simulink model "ACC_Controller"  (R2026b)
settings: Solver=FixedStepDiscrete  StopTime=inf  FixedStep=0.05
InitFcn:
  | acc_controller_init;
values from neighbouring files (symbols this model uses):
  C = acc_controller_params()    [acc_controller_init.m]    (also in acc_scenario_input.m; acc_scenarios.m; build_acc_controller.m; replay_mass_estimate.m)
libraries: mpclib x1
settings Model: Creator=kikiw  LastModifiedBy=kikiw
settings OptimizationCC: DefaultParameterBehavior=Inlined  DifferentSizesBufferReuse=on  EfficientTunableParamExpr=on  EnhancedBackFolding=on  OptimizationCustomize=off  OptimizeBlockOrder=speed  PassReuseOutputArgsAs=Individual arguments  RemoveInternalMemoryZeroInit=on  RemoveRootLevelIOMemoryZeroInit=on
settings DebuggingCC: ParameterTunabilityLossMsg=error
settings SFSimCC: MATLABDynamicMemAlloc=off
settings RTWCC: DataTypeReplacement=CDataTypesFixedWidth  Description=Embedded Coder  GenerateReport=on  SystemTargetFile=ert.tlc  TargetLang=C++  TemplateMakefile=ert_default_tmf
settings CodeAppCC: CustomSymbolStrUtil=$R$N$C  ForceParamTrailComments=on  IgnoreCustomStorageClasses=off  InsertBlockDesc=on  OperatorAnnotations=on  SFDataObjDesc=on  SimulinkDataObjDesc=on
settings ERTTargetCC: CodeInterfacePackaging=C++ class  CombineSignalStateStructs=on  GenerateSampleERTMain=on  MaxIdInt16=INT16_MAX  MaxIdInt32=INT32_MAX  MaxIdInt64=INT64_MAX  MaxIdInt8=INT8_MAX  MaxIdUint16=UINT16_MAX  MaxIdUint32=UINT32_MAX  MaxIdUint64=UINT64_MAX  MaxIdUint8=UINT8_MAX  MinIdInt16=INT16_MIN  MinIdInt32=INT32_MIN  MinIdInt64=INT64_MIN  MinIdInt8=INT8_MIN  RootIOFormat=Structure reference  SubcomponentCodeInterfacePackaging=C++ class  TargetLangStandard=C++11 (ISO)
settings CPPComponent: ExternalIOMemberVisibility=private  GenerateDestructor=on  GenerateExternalIOAccessMethods=Inlined structure-based method  GenerateInternalMemberAccessMethods=None  GenerateParameterAccessMethods=None  IncludeModelTypesInModelClass=on  InternalMemberVisibility=private  ParameterMemberVisibility=private  UseOperatorNewForModelRefRegistration=off

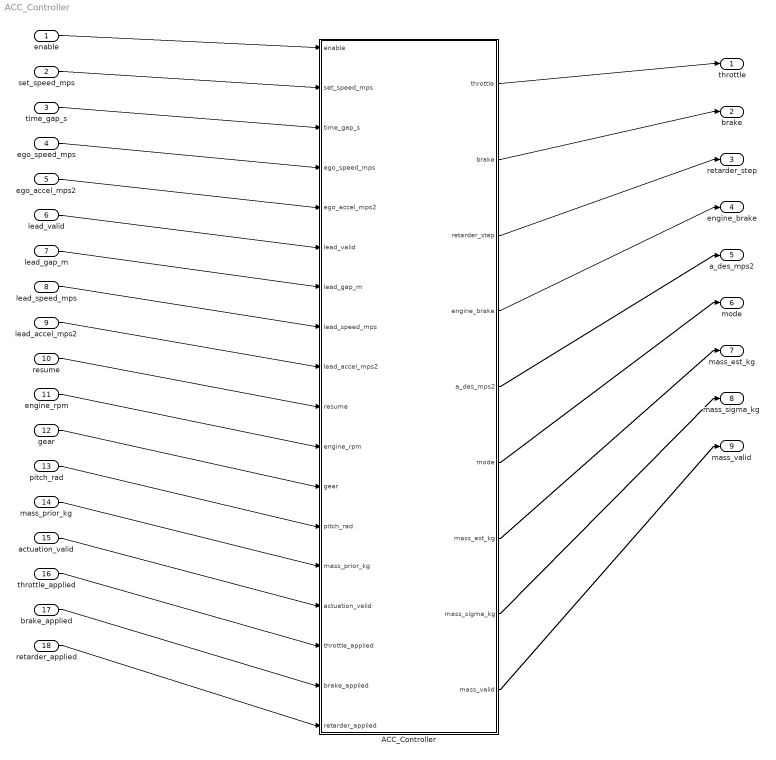
== system ACC_Controller ==
  enable : Inport  OutDataTypeStr=boolean  PortDimensions=1  SampleTime=C.Ts
  set_speed_mps : Inport  Port=2  OutDataTypeStr=double  PortDimensions=1  SampleTime=C.Ts
  time_gap_s : Inport  Port=3  OutDataTypeStr=double  PortDimensions=1  SampleTime=C.Ts
  ego_speed_mps : Inport  Port=4  OutDataTypeStr=double  PortDimensions=1  SampleTime=C.Ts
  ego_accel_mps2 : Inport  Port=5  OutDataTypeStr=double  PortDimensions=1  SampleTime=C.Ts
  lead_valid : Inport  Port=6  OutDataTypeStr=boolean  PortDimensions=1  SampleTime=C.Ts
  lead_gap_m : Inport  Port=7  OutDataTypeStr=double  PortDimensions=1  SampleTime=C.Ts
  lead_speed_mps : Inport  Port=8  OutDataTypeStr=double  PortDimensions=1  SampleTime=C.Ts
  lead_accel_mps2 : Inport  Port=9  OutDataTypeStr=double  PortDimensions=1  SampleTime=C.Ts
  resume : Inport  Port=10  OutDataTypeStr=boolean  PortDimensions=1  SampleTime=C.Ts
  engine_rpm : Inport  Port=11  OutDataTypeStr=double  PortDimensions=1  SampleTime=C.Ts
  gear : Inport  Port=12  OutDataTypeStr=int32  PortDimensions=1  SampleTime=C.Ts
  pitch_rad : Inport  Port=13  OutDataTypeStr=double  PortDimensions=1  SampleTime=C.Ts
  mass_prior_kg : Inport  Port=14  OutDataTypeStr=double  PortDimensions=1  SampleTime=C.Ts
  actuation_valid : Inport  Port=15  OutDataTypeStr=boolean  PortDimensions=1  SampleTime=C.Ts
  throttle_applied : Inport  Port=16  OutDataTypeStr=double  PortDimensions=1  SampleTime=C.Ts
  brake_applied : Inport  Port=17  OutDataTypeStr=double  PortDimensions=1  SampleTime=C.Ts
  retarder_applied : Inport  Port=18  OutDataTypeStr=int32  PortDimensions=1  SampleTime=C.Ts
  ACC_Controller : Subsystem  TreatAsAtomicUnit=on
  throttle : Outport  OutDataTypeStr=double
  brake : Outport  Port=2  OutDataTypeStr=double
  retarder_step : Outport  Port=3  OutDataTypeStr=int32
  engine_brake : Outport  Port=4  OutDataTypeStr=boolean
  a_des_mps2 : Outport  Port=5  OutDataTypeStr=double
  mode : Outport  Port=6  OutDataTypeStr=uint8
  mass_est_kg : Outport  Port=7  OutDataTypeStr=double
  mass_sigma_kg : Outport  Port=8  OutDataTypeStr=double
  mass_valid : Outport  Port=9  OutDataTypeStr=boolean
  wires:
  enable/1 -> ACC_Controller/1(enable)
  set_speed_mps/1 -> ACC_Controller/2(set_speed_mps)
  time_gap_s/1 -> ACC_Controller/3(time_gap_s)
  ego_speed_mps/1 -> ACC_Controller/4(ego_speed_mps)
  ego_accel_mps2/1 -> ACC_Controller/5(ego_accel_mps2)
  lead_valid/1 -> ACC_Controller/6(lead_valid)
  lead_gap_m/1 -> ACC_Controller/7(lead_gap_m)
  lead_speed_mps/1 -> ACC_Controller/8(lead_speed_mps)
  lead_accel_mps2/1 -> ACC_Controller/9(lead_accel_mps2)
  resume/1 -> ACC_Controller/10(resume)
  engine_rpm/1 -> ACC_Controller/11(engine_rpm)
  gear/1 -> ACC_Controller/12(gear)
  pitch_rad/1 -> ACC_Controller/13(pitch_rad)
  mass_prior_kg/1 -> ACC_Controller/14(mass_prior_kg)
  actuation_valid/1 -> ACC_Controller/15(actuation_valid)
  throttle_applied/1 -> ACC_Controller/16(throttle_applied)
  brake_applied/1 -> ACC_Controller/17(brake_applied)
  retarder_applied/1 -> ACC_Controller/18(retarder_applied)
  ACC_Controller/1(throttle) -> throttle/1
  ACC_Controller/2(brake) -> brake/1
  ACC_Controller/3(retarder_step) -> retarder_step/1
  ACC_Controller/4(engine_brake) -> engine_brake/1
  ACC_Controller/5(a_des_mps2) -> a_des_mps2/1
  ACC_Controller/6(mode) -> mode/1
  ACC_Controller/7(mass_est_kg) -> mass_est_kg/1
  ACC_Controller/8(mass_sigma_kg) -> mass_sigma_kg/1
  ACC_Controller/9(mass_valid) -> mass_valid/1

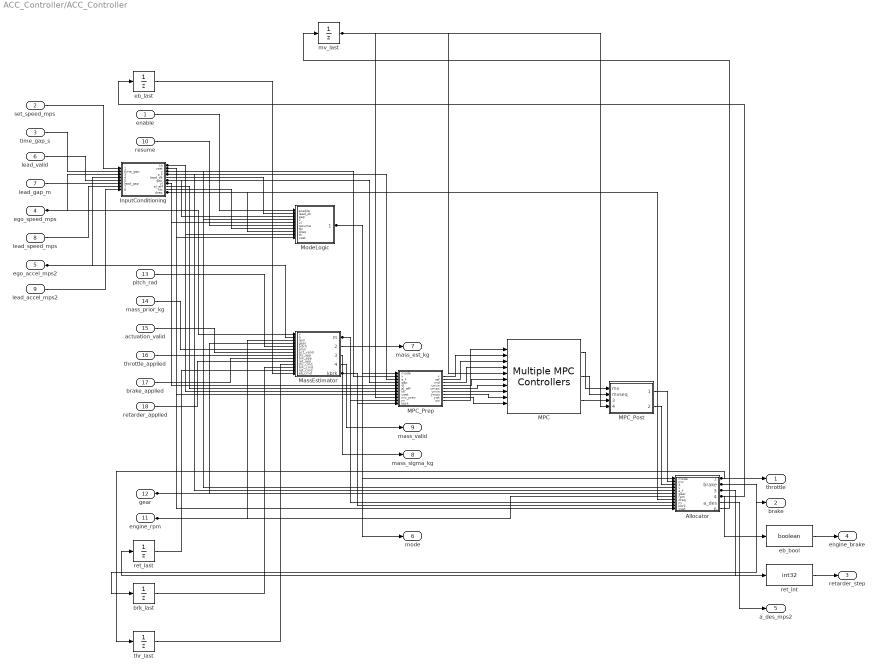
== system ACC_Controller/ACC_Controller ==
  enable : Inport
  set_speed_mps : Inport  Port=2
  time_gap_s : Inport  Port=3
  ego_speed_mps : Inport  Port=4
  ego_accel_mps2 : Inport  Port=5
  lead_valid : Inport  Port=6
  lead_gap_m : Inport  Port=7
  lead_speed_mps : Inport  Port=8
  lead_accel_mps2 : Inport  Port=9
  resume : Inport  Port=10
  engine_rpm : Inport  Port=11
  gear : Inport  Port=12
  pitch_rad : Inport  Port=13
  mass_prior_kg : Inport  Port=14
  actuation_valid : Inport  Port=15
  throttle_applied : Inport  Port=16
  brake_applied : Inport  Port=17
  retarder_applied : Inport  Port=18
  Allocator : MATLAB Function  TreatAsAtomicUnit=on
  InputConditioning : MATLAB Function  TreatAsAtomicUnit=on
  MPC : mpclib/Multiple MPC Controllers  mpcobjs={'mpcComfort','mpcEmergency'}  x0s={[],[]}  Nmpc=1  theMPC=1  nmv=1  nmo=1  nmd=1  nts=1  md_inport_multiple=on  mv_inport_multiple=on  uref_inport_multiple=off  return_cost_multiple=off  return_mvseq_multiple=on  return_qpstatus_multiple=on  return_xseq_multiple=off  return_state_multiple=off  return_ovseq_multiple=off  state_inport_multiple=on  umin_inport_multiple=on  umax_inport_multiple=on  ymin_inport_multiple=on  ymax_inport_multiple=on  ywt_inport_multiple=on  uwt_inport_multiple=off  duwt_inport_multiple=off  rhoeps_inport_multiple=off  BlockDataType_multiple=double  SampleTimeInherited_multiple=off
  MPC_Post : MATLAB Function  TreatAsAtomicUnit=on
  MPC_Prep : MATLAB Function  TreatAsAtomicUnit=on
  MassEstimator : MATLAB Function  TreatAsAtomicUnit=on
  ModeLogic : Stateflow chart  TreatAsAtomicUnit=on
  brk_last : UnitDelay  SampleTime=C.Ts
  eb_bool : DataTypeConversion  OutDataTypeStr=boolean  SaturateOnIntegerOverflow=off  RndMeth=Floor
  eb_last : UnitDelay  InitialCondition=false  SampleTime=C.Ts
  mv_last : UnitDelay  InitialCondition=[0; 0]  SampleTime=C.Ts
  ret_int : DataTypeConversion  OutDataTypeStr=int32  SaturateOnIntegerOverflow=off  RndMeth=Floor
  ret_last : UnitDelay  SampleTime=C.Ts
  thr_last : UnitDelay  SampleTime=C.Ts
  throttle : Outport
  brake : Outport  Port=2
  retarder_step : Outport  Port=3
  engine_brake : Outport  Port=4
  a_des_mps2 : Outport  Port=5
  mode : Outport  Port=6
  mass_est_kg : Outport  Port=7
  mass_sigma_kg : Outport  Port=8
  mass_valid : Outport  Port=9
  wires:
  MPC_Prep/9(sw) -> MPC/1
  MassEstimator/2(mass_est) -> mass_est_kg/1
  enable/1 -> ModeLogic/1(enable)
  set_speed_mps/1 -> InputConditioning/1(set_speed)
  time_gap_s/1 -> InputConditioning/2(time_gap)
  ego_speed_mps/1 -> MassEstimator/1(v), InputConditioning/3(ego_speed)
  eb_bool/1 -> engine_brake/1
  lead_valid/1 -> InputConditioning/5(lead_valid)
  lead_gap_m/1 -> InputConditioning/6(lead_gap)
  lead_speed_mps/1 -> InputConditioning/7(lead_speed)
  ego_accel_mps2/1 -> MassEstimator/2(a), InputConditioning/4(ego_accel)
  engine_rpm/1 -> Allocator/7(rpm), MassEstimator/3(rpm)
  gear/1 -> Allocator/6(gear), MassEstimator/4(gear)
  resume/1 -> ModeLogic/6(resume)
  lead_accel_mps2/1 -> InputConditioning/8(lead_accel)
  Allocator/5(a_des) -> a_des_mps2/1
  MassEstimator/1(m) -> Allocator/9(m), MPC_Prep/10(m)
  eb_last/1 -> MassEstimator/14(eb_cmd)
  InputConditioning/1(th) -> MPC_Prep/7(th), ModeLogic/9(th)
  InputConditioning/2(vset) -> Allocator/11(vset), MPC_Prep/8(vset), ModeLogic/10(vset)
  InputConditioning/3(v) -> MPC_Prep/2(v), Allocator/4(v), ModeLogic/4(v)
  InputConditioning/4(a_f) -> Allocator/5(a_f), MPC_Prep/3(a_f)
  MPC/2 -> MPC_Post/2(mvseq)
  InputConditioning/5(lead_ok) -> ModeLogic/2(lead_ok)
  InputConditioning/6(gap) -> MPC_Prep/4(gap), ModeLogic/3(gap)
  InputConditioning/7(vl) -> MPC_Prep/5(vl), ModeLogic/5(vl)
  retarder_applied/1 -> MassEstimator/10(ret_app)
  brake_applied/1 -> MassEstimator/9(brk_app)
  InputConditioning/8(al_eff) -> MPC_Prep/6(al_eff)
  InputConditioning/9(ttc) -> ModeLogic/7(ttc)
  InputConditioning/10(dreq) -> Allocator/8(dreq), ModeLogic/8(dreq)
  throttle_applied/1 -> MassEstimator/8(thr_app)
  actuation_valid/1 -> MassEstimator/7(act_valid)
  mass_prior_kg/1 -> MassEstimator/6(prior)
  pitch_rad/1 -> MassEstimator/5(pitch)
  ret_last/1 -> MassEstimator/13(ret_cmd)
  brk_last/1 -> MassEstimator/12(brk_cmd)
  MPC_Post/1(mv_used) -> Allocator/2(mv)
  thr_last/1 -> MassEstimator/11(thr_cmd)
  MPC/3 -> MPC_Post/3(qp_status)
  mv_last/1 -> MPC_Post/4(mv_prev), MPC/5, MPC_Prep/9(mv_prev)
  ModeLogic/1(mode) -> Allocator/1(mode), MPC_Prep/1(mode), mode/1
  MPC_Prep/7(ymax) -> MPC/9
  MassEstimator/3(mass_sigma) -> mass_sigma_kg/1
  MPC_Prep/5(umax) -> MPC/7
  MassEstimator/4(mass_valid) -> mass_valid/1
  MassEstimator/5(kbrk) -> Allocator/10(kbrk), MPC_Prep/11(kbrk)
  MPC_Prep/1(x) -> MPC/2
  MPC_Prep/2(ref) -> MPC/3
  MPC_Prep/3(md) -> MPC/4
  MPC_Prep/4(umin) -> MPC/6
  MPC_Prep/6(ymin) -> MPC/8
  Allocator/6(mv_app) -> mv_last/1
  MPC_Prep/8(ywt) -> MPC/10
  MPC_Post/2(a_seq_mean) -> Allocator/3(a_seq_mean)
  MPC/1 -> MPC_Post/1(mv)
  Allocator/1(throttle) -> thr_last/1, throttle/1
  Allocator/2(brake) -> brk_last/1, brake/1
  Allocator/3(ret_step) -> ret_int/1, ret_last/1
  Allocator/4(engine_brake) -> eb_last/1, eb_bool/1
  ret_int/1 -> retarder_step/1

== matlab function ACC_Controller/InputConditioning ==
  data: set_speed input; th output; time_gap input; ego_speed input; ego_accel input; lead_valid input; lead_gap input; lead_speed input; lead_accel input; vset output; v output; a_f output; lead_ok output; gap output; vl output; al_eff output; ttc output; dreq output; C parameter
function [th, vset, v, a_f, lead_ok, gap, vl, al_eff, ttc, dreq] = InputConditioning(set_speed, time_gap, ego_speed, ego_accel, lead_valid, lead_gap, lead_speed, lead_accel, C)
[th, vset, v, a_f, lead_ok, gap, vl, al_eff, ttc, dreq] = acc_condition(set_speed, time_gap, ego_speed, ego_accel, lead_valid, lead_gap, lead_speed, lead_accel, C);

== stateflow chart ACC_Controller/ModeLogic ==
  settings: updateMethod=DISCRETE  sampleTime=0.05  description=ACC modes: 0 OFF, 1 CRUISE, 2 FOLLOW, 3 STOP, 4 HOLD, 5 GO, 6 EMERGENCY. enable false -> OFF. FOLLOW when a lead is within the follow range; STOP when the lead has stopped; HOLD at standstill (brake held); GO automatically when the lead pulls away by more than MODE_go_gap within MODE_go_window s of stopping, otherwise on resume; EMERGENCY when TTC < MODE_ttc_on or the required deceleration > MODE_dreq_on. A set speed below MODE_vset_stop is a stop request: CRUISE / FOLLOW / GO go to HOLD at standstill, HOLD does not go to GO and returns to CRUISE if the driver pushes the truck above MODE_hold_release_v.
  state OFF
    entry: mode = uint8(0);
  state ON
    state CRUISE
      entry: mode = uint8(1);
    state FOLLOW
      entry: mode = uint8(2);
    state STOP
      entry: mode = uint8(3);
    state GO
      entry: mode = uint8(5);
    state HOLD
      entry: mode = uint8(4);
      during: t_hold = t_hold + MODE_dt;
    state EMERGENCY
      entry: mode = uint8(6);
    STOP -> CRUISE [order 4] : [duration(~lead_ok) > MODE_lead_lost_s]
    STOP -> FOLLOW [order 3] : [lead_ok && vl > MODE_v_lead_moving]
    FOLLOW -> CRUISE [order 3] : [duration(~lead_ok) > MODE_lead_lost_s || (lead_ok && gap > follow_range() + MODE_follow_hyst)]
    FOLLOW -> EMERGENCY [order 1] : [lead_ok && (ttc < MODE_ttc_on || dreq > MODE_dreq_on)]
    STOP -> EMERGENCY [order 1] : [lead_ok && (ttc < MODE_ttc_on || dreq > MODE_dreq_on)]
    (junction 46) -> CRUISE [order 3]
    HOLD -> CRUISE [order 2] : [vset < MODE_vset_stop && v > MODE_hold_release_v]
    EMERGENCY -> CRUISE [order 3] : [duration(~lead_ok) > MODE_emerg_hold]
    GO -> CRUISE [order 4] : [v > MODE_go_done_v && ~lead_ok]
    (junction 46) -> FOLLOW [order 2] : [lead_ok && gap < follow_range()]
    EMERGENCY -> FOLLOW [order 2] : [lead_ok && duration(ttc > MODE_ttc_off && dreq < MODE_dreq_off) > MODE_emerg_hold]
    CRUISE -> FOLLOW [order 2] : [lead_ok && gap < follow_range()]
    GO -> FOLLOW [order 3] : [v > MODE_go_done_v && lead_ok]
    GO -> STOP [order 2] : [lead_ok && vl < MODE_v_lead_stopped && v < MODE_v_lead_moving]
    FOLLOW -> STOP [order 2] : [lead_ok && vl < MODE_v_lead_stopped]
    STOP -> HOLD [order 2] : [v < MODE_v_standstill]{t_hold = 0; gap_stop = gap;}
    CRUISE -> EMERGENCY [order 1] : [lead_ok && (ttc < MODE_ttc_on || dreq > MODE_dreq_on)]
    CRUISE -> HOLD [order 3] : [vset < MODE_vset_stop && v < MODE_v_standstill]{t_hold = 99; gap_stop = gap;}
    FOLLOW -> HOLD [order 4] : [vset < MODE_vset_stop && v < MODE_v_standstill]{t_hold = 99; gap_stop = gap;}
    (default) -> (junction 46)
    (junction 46) -> HOLD [order 1] : [v < MODE_v_standstill]{t_hold = 99; gap_stop = gap;}
    HOLD -> GO [order 1] : [vset >= MODE_vset_stop && (resume || (t_hold <= MODE_go_window && lead_ok && gap > gap_stop + MODE_go_gap))]
    GO -> EMERGENCY [order 1] : [lead_ok && (ttc < MODE_ttc_on || dreq > MODE_dreq_on)]
    EMERGENCY -> HOLD [order 1] : [v < MODE_v_standstill]{t_hold = 0; gap_stop = gap;}
    GO -> HOLD [order 5] : [vset < MODE_vset_stop && v < MODE_v_standstill]{t_hold = 99; gap_stop = gap;}
  (default) -> OFF
  ON -> OFF : [~enable]
  OFF -> ON : [enable]
  data: r function_output; enable input size=1; lead_ok input size=1; gap input size=1; v input size=1; vl input size=1; resume input size=1; ttc input size=1; dreq input size=1; th input size=1; vset input size=1; mode output uint8 =0; t_hold local =99; gap_stop local =0; MODE_follow_range_extra parameter; MODE_follow_preview_s parameter; MODE_follow_hyst parameter; MODE_lead_lost_s parameter; MODE_v_lead_stopped parameter; MODE_v_lead_moving parameter; MODE_v_standstill parameter; MODE_go_gap parameter; MODE_go_window parameter; MODE_go_done_v parameter; MODE_ttc_on parameter; MODE_dreq_on parameter; MODE_ttc_off parameter; MODE_dreq_off parameter; MODE_emerg_hold parameter; MODE_vset_stop parameter; MODE_hold_release_v parameter; MODE_dt parameter; FOL_d0 parameter; FOL_a_approach parameter; FOL_k_gap parameter
  function r = follow_range:
    | function r = follow_range()
    | % distance within which a lead matters: target gap + error at which the approach profile
    | % starts at this closing speed (acc_mpc_prep) + the closing distance over the preview + margin
    | vr = max(v - vl, 0);
    | c = FOL_a_approach / FOL_k_gap;
    | r = FOL_d0 + th*v + vr*(vr + 2*c)/(2*FOL_a_approach) + MODE_follow_preview_s*vr + MODE_follow_range_extra;

== matlab function ACC_Controller/MPC_Prep ==
  data: mode input; x output; v input; a_f input; gap input; vl input; al_eff input; th input; vset input; mv_prev input; m input; kbrk input; ref output; md output; umin output; umax output; ymin output; ymax output; ywt output; sw output; C parameter
function [x, ref, md, umin, umax, ymin, ymax, ywt, sw] = MPC_Prep(mode, v, a_f, gap, vl, al_eff, th, vset, mv_prev, m, kbrk, C)
[x, ref, md, umin, umax, ymin, ymax, ywt, sw] = acc_mpc_prep(double(mode), v, a_f, gap, vl, al_eff, th, vset, mv_prev, m, kbrk, C);

== matlab function ACC_Controller/MPC_Post ==
  data: mv input; mv_used output; mvseq input; qp_status input; mv_prev input; a_seq_mean output; C parameter
function [mv_used, a_seq_mean] = MPC_Post(mv, mvseq, qp_status, mv_prev, C)
% QP failure (status < 0: infeasible or numerical): never accelerate, keep the last braking
if qp_status < 0
    mv_used = [min(mv_prev(1), 0); mv_prev(2)];
else
    mv_used = mv;
end
% mean of the predicted total request (drive + brake path) over C.alc.ret5_window
n = min(size(mvseq, 1), max(1, round(C.alc.ret5_window / C.Ts)));
a_seq_mean = sum(sum(mvseq(1:n, :))) / n;

== matlab function ACC_Controller/Allocator ==
  data: mode input; throttle output double size=1; mv input; a_seq_mean input; v input; a_f input; gear input; rpm input; dreq input; m input; kbrk input; vset input; brake output double size=1; ret_step output double size=1; engine_brake output boolean size=1; a_des output double size=1; mv_app output double size=[2 1]; C parameter
function [throttle, brake, ret_step, engine_brake, a_des, mv_app] = Allocator(mode, mv, a_seq_mean, v, a_f, gear, rpm, dreq, m, kbrk, vset, C)
[throttle, brake, ret_step, engine_brake, a_des, mv_app] = acc_allocate(double(mode), mv, a_seq_mean, v, a_f, gear, rpm, dreq, m, kbrk, vset, C);

== matlab function ACC_Controller/MassEstimator ==
  data: v input; m output double size=1; a input; rpm input; gear input; pitch input; prior input; act_valid input; thr_app input; brk_app input; ret_app input; thr_cmd input; brk_cmd input; ret_cmd input; eb_cmd input; mass_est output double size=1; mass_sigma output double size=1; mass_valid output boolean size=1; kbrk output double size=1; C parameter
function [m, mass_est, mass_sigma, mass_valid, kbrk] = MassEstimator(v, a, rpm, gear, pitch, prior, act_valid, thr_app, brk_app, ret_app, thr_cmd, brk_cmd, ret_cmd, eb_cmd, C)
% applied pedals / retarder step from the harness when actuation_valid, else the controller's
% own commands of the previous step
thr = thr_cmd; brk = brk_cmd; ret = ret_cmd;
if act_valid && isfinite(thr_app), thr = thr_app; end
if act_valid && isfinite(brk_app), brk = brk_app; end
if act_valid && ret_app >= 0, ret = double(ret_app); end
[m, mass_est, mass_sigma, mass_valid, kbrk] = acc_mass_estimate(v, a, rpm, double(gear), thr, brk, ret, logical(eb_cmd), pitch, prior, C);
